simulink model "HW1_matlab"  (R2023b)
settings: Solver=VariableStepAuto  StartTime=0.0  StopTime=10.0  RelTol=1e-3
model workspace (MAT data in the model file):
  b = 128
libraries: commdigbbndam3 x3, commchan3 x2, commsink2 x2, dspxfrm3 x2, commrandsrc3 x1
settings Model: Creator=chang  LastModifiedBy=chang

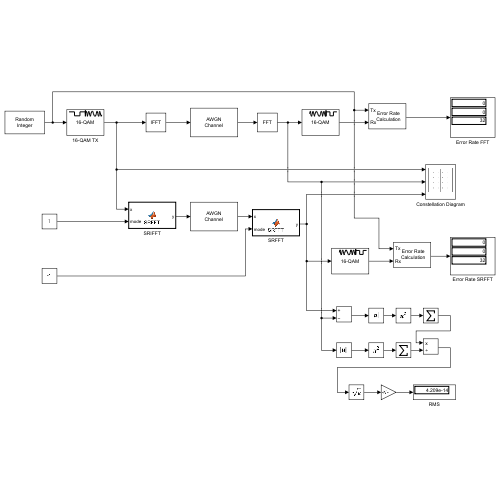
[thumbnail: Simulink's stored preview of the top-level diagram]
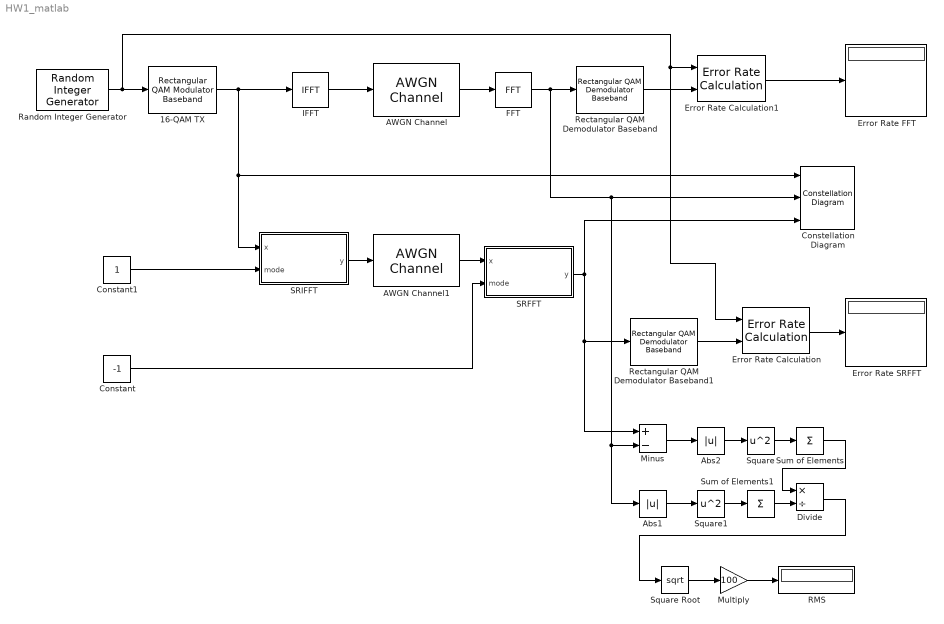
== system HW1_matlab ==
  16-QAM TX : commdigbbndam3/Rectangular QAM Modulator Baseband  M=16  InType=Integer  Enc=Gray  Mapping=[0:15]  PowType=Average Power  MinDist=2  AvgPow=1  PeakPow=1  Ph=0  outDtype=double  outWordLen=16  outUDDataType=sfix(16)  outFracLenMode=Best precision  outFracLen=15  outDataTypeStr=double  outLastDataTypeStr=double
  AWGN Channel : commchan3/AWGN Channel  LegacyMode=on  NoiseMethod="Signal to noise ratio  (SNR)"  noiseMode="Signal to noise ratio  (Eb/No)"  EbNo=40  EsNo=10  SNR=10  BitsPerSymbol=2  SignalPower=1  SamplesPerSymbol=1  SymbolPeriod=1  VarianceSource=Parameter  Variance=1  RandomStream=Global stream  Seed=70  SimulateUsing=Code generation
  AWGN Channel1 : commchan3/AWGN Channel  LegacyMode=on  NoiseMethod="Signal to noise ratio  (SNR)"  noiseMode="Signal to noise ratio  (Eb/No)"  EbNo=40  EsNo=10  SNR=10  BitsPerSymbol=2  SignalPower=1  SamplesPerSymbol=1  SymbolPeriod=1  VarianceSource=Parameter  Variance=1  RandomStream=Global stream  Seed=70  SimulateUsing=Code generation
  Abs1 : Abs  SaturateOnIntegerOverflow=off
  Abs2 : Abs  SaturateOnIntegerOverflow=off
  Constant : Constant  Value=-1
  Constant1 : Constant
  Constellation Diagram : ConstellationDiagram  NumInputPorts=3  WindowPosition=[1739.000000,459.000000,600.000000,600.000000,]  Visible=on  ScopeFrameLocation=window  ReferenceConstellation="{[0.7071+0.7071i          -0.7071+0.7071i          -0.7071-0.7071i            0.707-0.7071i][0.7071+0.7071i          -0.7071+0.7071i          -0.7071-0.7071i            0.707-0.7071i][0.7071+0.7071i          -0.7071+0.7071i          -0.7071-0.7071i            0.707-0.7071i]}"  ShowLegend=on
  Divide : Product  Inputs=*/
  Error Rate Calculation : commsink2/Error Rate Calculation  N=0  st_delay=0  cp_mode=Entire frame  subframe=[]  PMode=Port  WsName=ErrorVec  RsMode2=off  stop=off  numErr=100  maxBits=1e6
  Error Rate Calculation1 : commsink2/Error Rate Calculation  N=0  st_delay=0  cp_mode=Entire frame  subframe=[]  PMode=Port  WsName=ErrorVec  RsMode2=off  stop=off  numErr=100  maxBits=1e6
  Error Rate FFT : Display
  Error Rate SRFFT : Display
  FFT : dspxfrm3/FFT  FFTImplementation=Auto  CompMethod=Table lookup  TableOpt=NEW  TableOptActive=Speed  BitRevOrder=off  Normalize=off  InheritFFTLength=on  FFTLength=64  WrapInput=on  roundingMode=Floor  overflowMode=off  firstCoeffDataTypeStr=Inherit: Same word length as input  firstCoeffLastDataTypeStr=Inherit: Same word length as input  outputMin=[]  outputMax=[]
  IFFT : dspxfrm3/IFFT  FFTImplementation=Auto  CompMethod=Table lookup  TableOpt=NEW  TableOptActive=Speed  BitRevOrder=off  cs_in=off  Normalize=on  InheritFFTLength=on  FFTLength=64  WrapInput=on  mode=Complex  outSamplingMode=Sample based  roundingMode=Floor  overflowMode=off  firstCoeffDataTypeStr=Inherit: Same word length as input  firstCoeffLastDataTypeStr=Inherit: Same word length as input  outputMin=[]  outputMax=[]
  Minus : Sum  Inputs=+-
  Multiply : Gain  Gain=100
  RMS : Display
  Random Integer Generator : commrandsrc3/Random Integer Generator  SetSize=16  SeedSource=Parameter  Seed=37  SampleTime=1  SamplesPerFrame=32  OutputDataType=double  SimulateUsing=Interpreted execution
  Rectangular QAM Demodulator Baseband : commdigbbndam3/Rectangular QAM Demodulator Baseband  M=16  OutType=Integer  DecType=Hard decision  VarSource=Dialog  Variance=1  Dec=Gray  Mapping=[0:15]  PowType=Average Power  MinDist=2  AvgPow=1  PeakPow=1  Ph=0  outDtype1=Inherit via internal rule  outDtype2=Inherit via internal rule  derotateFactorWordLen=16  derotateFactorDataTypeStr=Inherit: Same word length as input  derotateFactorLastDataTypeStr=Inherit: Same word length as input  denormFactorWordLen=16  denormFactorDataTypeStr=Inherit: Same word length as input  denormFactorLastDataTypeStr=Inherit: Same word length as input  prodOutWordLen=32  prodOutOverflowMode=Wrap  prodOutRoundingMode=Floor  prodOutOvFlMode=off  prodOutOvFlModeLastStrValue=off  sumWordLen=32
  Rectangular QAM Demodulator Baseband1 : commdigbbndam3/Rectangular QAM Demodulator Baseband  M=16  OutType=Integer  DecType=Hard decision  VarSource=Dialog  Variance=1  Dec=Gray  Mapping=[0:15]  PowType=Average Power  MinDist=2  AvgPow=1  PeakPow=1  Ph=0  outDtype1=Inherit via internal rule  outDtype2=Inherit via internal rule  derotateFactorWordLen=16  derotateFactorDataTypeStr=Inherit: Same word length as input  derotateFactorLastDataTypeStr=Inherit: Same word length as input  denormFactorWordLen=16  denormFactorDataTypeStr=Inherit: Same word length as input  denormFactorLastDataTypeStr=Inherit: Same word length as input  prodOutWordLen=32  prodOutOverflowMode=Wrap  prodOutRoundingMode=Floor  prodOutOvFlMode=off  prodOutOvFlModeLastStrValue=off  sumWordLen=32
  SRFFT : MATLAB Function  TreatAsAtomicUnit=on
  SRIFFT : MATLAB Function  TreatAsAtomicUnit=on
  Square : Math  Operator=square
  Square Root : Sqrt
  Square1 : Math  Operator=square
  Sum of Elements : Sum  Inputs=+
  Sum of Elements1 : Sum  Inputs=+
  wires:
  AWGN Channel/1 -> FFT/1
  16-QAM TX/1 -> IFFT/1, SRIFFT/1(x), Constellation Diagram/1
  IFFT/1 -> AWGN Channel/1
  FFT/1 -> Abs1/1, Minus/2, Constellation Diagram/2, Rectangular QAM Demodulator Baseband/1
  Random Integer Generator/1 -> Error Rate Calculation/1, Error Rate Calculation1/1, 16-QAM TX/1
  Constant/1 -> SRFFT/2(mode)
  SRFFT/1(y) -> Minus/1, Rectangular QAM Demodulator Baseband1/1, Constellation Diagram/3
  Constant1/1 -> SRIFFT/2(mode)
  Error Rate Calculation/1 -> Error Rate SRFFT/1
  AWGN Channel1/1 -> SRFFT/1(x)
  SRIFFT/1(y) -> AWGN Channel1/1
  Error Rate Calculation1/1 -> Error Rate FFT/1
  Rectangular QAM Demodulator Baseband1/1 -> Error Rate Calculation/2
  Rectangular QAM Demodulator Baseband/1 -> Error Rate Calculation1/2
  Square Root/1 -> Multiply/1
  Divide/1 -> Square Root/1
  Square1/1 -> Sum of Elements1/1
  Sum of Elements/1 -> Divide/1
  Minus/1 -> Abs2/1
  Square/1 -> Sum of Elements/1
  Abs1/1 -> Square1/1
  Sum of Elements1/1 -> Divide/2
  Abs2/1 -> Square/1
  Multiply/1 -> RMS/1

== matlab function HW1_matlab/SRFFT ==
  data: x input; y output; mode input
function y = SRFFT(x,mode)


N = length(x);
log2n = log2(N);

x = bitrevorder(x);

for stage = 1 : log2n
    group_member = 2^(stage); 
    node_spacing = group_member/2;
    wm = twiddle_factor(1,group_member,mode);
    % Group Loop
    for index = 0 : group_member : N-1
        w= 1.0+0.0j;
        % Butterfly Loop
        for k= 0 : node_spacing-1
            t = x(index+k+node_spacing+1)*w;
            u = x(index+k+1);
            x(index+k+1) = u + t;
            x(index+k+node_spacing+1) = u - t;
            w = w*wm;
        end
    end
end
if (mode == 1)
    y=x/N;
else
    y=x;
end

function y = twiddle_factor(k,n,mode)
% mode -1 --> FFT
% mode 1 --> IFFT

if (k==0)
    y = 1;
elseif (k * 4 == n)
    if (mode == -1)
        y = -1i;
    else
        y = 1i;
    end
elseif (k * 2 == n)
    y = -1.0;
elseif (k * 4 == 3* n)
    if (mode == -1)
        y = 1i;
    else
        y = -1i;
    end
else
    angle = mode * 2 * pi * k/n;
    y = exp(1i*angle);
end

== matlab function HW1_matlab/SRIFFT ==
  data: x input; y output; mode input
function y = SRFFT(x,mode)


N = length(x);
log2n = log2(N);

x = bitrevorder(x);

for stage = 1 : log2n
    group_member = 2^(stage); 
    node_spacing = group_member/2;
    wm = twiddle_factor(1,group_member,mode);
    % Group Loop
    for index = 0 : group_member : N-1
        w= 1.0+0.0j;
        % Butterfly Loop
        for k= 0 : node_spacing-1
            t = x(index+k+node_spacing+1)*w;
            u = x(index+k+1);
            x(index+k+1) = u + t;
            x(index+k+node_spacing+1) = u - t;
            w = w*wm;
        end
    end
end
if (mode == 1)
    y=x/N;
else
    y=x;
end

function y = twiddle_factor(k,n,mode)
% mode -1 --> FFT
% mode 1 --> IFFT

if (k==0)
    y = 1;
elseif (k * 4 == n)
    if (mode == -1)
        y = -1i;
    else
        y = 1i;
    end
elseif (k * 2 == n)
    y = -1.0;
elseif (k * 4 == 3* n)
    if (mode == -1)
        y = 1i;
    else
        y = -1i;
    end
else
    angle = mode * 2 * pi * k/n;
    y = exp(1i*angle);
end
